simulink model "traj_controller_mass_point_example"  (R2018b)
settings: Solver=ode1  StartTime=0.0  StopTime=80  FixedStep=0.001  RelTol=1e-3
values from neighbouring files (symbols this model uses):
  cycle = true    [traj_controller_mass_point_example_init.m]    (also in traj_from_waypoints_example.m = false; traj_rigid_body_example_init.m)
  inital_velo = 8    [traj_controller_mass_point_example_init.m]    (also in traj_from_waypoints_example.m = 15; traj_rigid_body_example_init.m = 20)
  traj = trajFromWaypoints(traj_empty, waypoints, degree, cycle)    [traj_controller_mass_point_example_init.m]    (also in traj_from_waypoints_example.m = trajFromWaypoints(traj, waypoints, degree, cycle); traj_rigid_body_example_init.m)
  waypoints = [1 -1 0.2; 2 0 0.1; 1 1 0; -1 -1 0; -2 0 0.1; -1 1 0.2]'*50    [traj_controller_mass_point_example_init.m]    (also in traj_from_waypoints_example.m = [1 1 1; 2 2 2; 3 3 3; 4 4 4]'; traj_rigid_body_example_init.m)
libraries: actuators_lib x2, rigidBody_lib x1, simulink x1, traj_lib x1
settings Model: Creator=Fgücker  LastModifiedBy=yannic

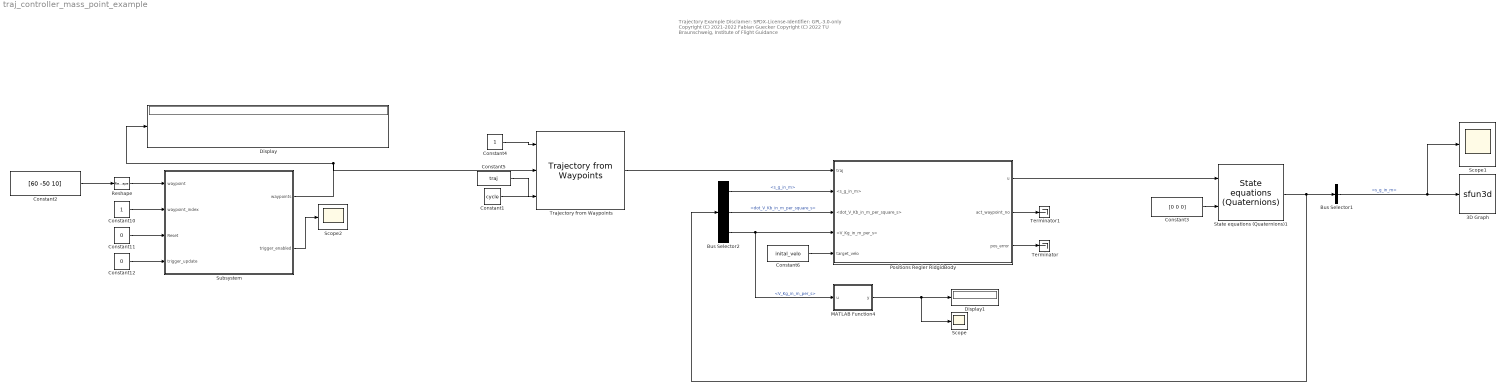
== system traj_controller_mass_point_example ==
  note: Trajectory Example
      |
      | Disclamer:
      | SPDX-License-Identifier: GPL-3.0-only
      |
      | Copyright (C) 2021-2022 Fabian Guecker
      | Copyright (C) 2022 TU Braunschweig, Institute of Flight Guidance
  3D Graph : S-Function  LoadFcn=if exist('sfun3d','file'), sfun3d([],[],[],'LoadBlock'); end  FunctionName=sfun3d  Parameters=ax,T,np,cp,gd,ls,mk,mx,hd,tb  SFunctionDeploymentMode=off  EnableBusSupport=off  mask(3D Graph){np=1, ax=[-1 1 -1 1 -1 1]*300, mx=1e4, T=0.040, cp=[0 0 1]*20, gd=on, hd=off, tb=off, ls=-, mk=none}
      mask prompts: np "Number of moving points (lines)"; ax "Range: [xmin xmax  ymin ymax zmin zmax]"; mx "Max number of points in each line"; T "Sampling Time"; cp "Camera position (use [0 0 1] for 2D XY view)"; gd "Grid (on|off)"; hd "HeadMarkers (on|off)"; tb "Toolbar (on|off)"; ls "LineStyle"; mk "LineMarker"
      mask help:
      | This block plots the position of several points in the XYZ space. The input contains the coordinates of all the points (x1,y1,z1,x2,y2,z2,...).
      | The number of moving points (lines), the XYZ ranges, sampling time, camera position, and grid (among other things) can be set as mask parameters.
      settings: CopyFcn=if exist('sfun3d','file'), sfun3d([],[],[],'CopyBlock'); end  DeleteFcn=if exist('sfun3d','file'), sfun3d([],[],[],'DeleteBlock'); end  NameChangeFcn=if exist('sfun3d','file'), sfun3d([],[],[],'NameChange'); end
      mask Help:
      | This block plots the position of several points in the XYZ space. The input contains the coordinates of all the points (x1,y1,z1,x2,y2,z2,...).
      | The number of moving points (lines), the XYZ ranges, sampling time, camera position, and grid (among other things) can be set as mask parameters.
      mask TypeOptions ls: - | -- | : | -. | none
      mask TypeOptions mk: none | . | + | o | * | x | square | diamond | v | ^ | > | < | pentagram | hexagram
      mask Display: plot([.05 .95 .95 .05 .05],[.45 .45 .95 .95 .45], 0.5+cos(0:0.1:2*pi)*0.3,0.7+sin(0:0.1:2*pi)*0.2)
  Bus Selector1 : BusSelector  OutputSignals=s_g_in_m
  Bus Selector2 : BusSelector  OutputSignals=s_g_in_m,dot_V_Kb_in_m_per_square_s,V_Kg_in_m_per_s
  Constant1 : Constant  Value=cycle  OutDataTypeStr=boolean
  Constant10 : Constant
  Constant11 : Constant  Value=0
  Constant12 : Constant  Value=0
  Constant2 : Constant  Value=[60 -50 10]
  Constant3 : Constant  Value=[0 0 0]
  Constant4 : Constant  OutDataTypeStr=boolean
  Constant5 : Constant  Value=traj  OutDataTypeStr=Bus: trajectoryBus
  Constant6 : Constant  Value=inital_velo
  Display : Display
  Display1 : Display
  MATLAB Function4 : MATLAB Function  TreatAsAtomicUnit=on
  Positions Regler RidgidBody : Subsystem
  Reshape : Reshape  OutputDimensionality=Column vector (2-D)
  Scope : Scope
  Scope1 : Scope
  Scope2 : Scope
  State equations (Quaternions)1 : rigidBody_lib/State equations (Quaternions)  m=1  I=eye(3)  g=9.81  omega_Kb_0=[0,0,0]'  q_bg_0=[1,0,0,0]'  V_Kb_0=inital_vel_vec  s_g_0=inital_point
  Subsystem : Subsystem  mask{MaxNumWaypoints=6}
      mask prompts: MaxNumWaypoints "Max. number of waypoints"
  Terminator : Terminator
  Terminator1 : Terminator
  Trajectory from Waypoints : traj_lib/Trajectory from Waypoints  traj_params=traj_params
      settings: SourceProductName=LADAC
  wires:
  Constant3/1 -> State equations (Quaternions)1/2
  State equations (Quaternions)1/1 -> Bus Selector1/1, Bus Selector2/1
  Bus Selector1/1 -> Scope1/1, 3D Graph/1  "<s_g_in_m>"
  Constant2/1 -> Reshape/1
  Subsystem/2(trigger_enabled) -> Scope2/1
  Subsystem/1(waypoints) -> Trajectory from Waypoints/2, Display/1
  Constant10/1 -> Subsystem/2(waypoint_index)
  Constant11/1 -> Subsystem/3(Reset)
  Constant12/1 -> Subsystem/4(trigger_update)
  Constant4/1 -> Trajectory from Waypoints/1
  Trajectory from Waypoints/1 -> Positions Regler RidgidBody/1(traj)
  Bus Selector2/1 -> Positions Regler RidgidBody/2(<s_g_in_m>)  "<s_g_in_m>"
  Bus Selector2/2 -> Positions Regler RidgidBody/3(<dot_V_Kb_in_m_per_square_s>)  "<dot_V_Kb_in_m_per_square_s>"
  Bus Selector2/3 -> MATLAB Function4/1(u), Positions Regler RidgidBody/4(<V_Kg_in_m_per_s>)  "<V_Kg_in_m_per_s>"
  Positions Regler RidgidBody/1(u) -> State equations (Quaternions)1/1
  Constant6/1 -> Positions Regler RidgidBody/5(target_velo)
  Positions Regler RidgidBody/3(pos_error) -> Terminator/1
  Positions Regler RidgidBody/2(act_waypoint_no) -> Terminator1/1
  MATLAB Function4/1(y) -> Scope/1, Display1/1
  Reshape/1 -> Subsystem/1(waypoint)
  Constant1/1 -> ?
  Constant5/1 -> Trajectory from Waypoints/3

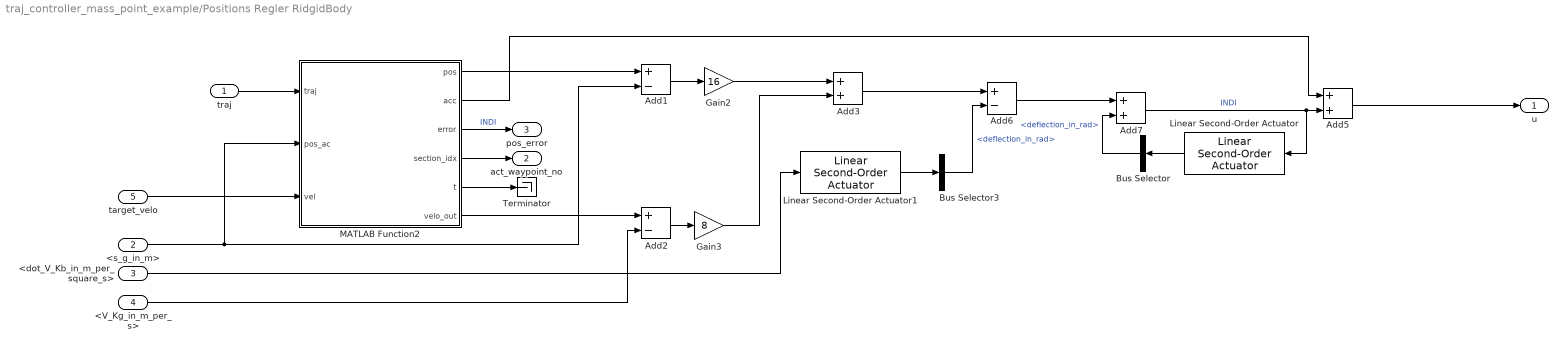
== system traj_controller_mass_point_example/Positions Regler RidgidBody ==
  traj : Inport
  <s_g_in_m> : Inport  Port=2
  <dot_V_Kb_in_m_per_square_s> : Inport  Port=3
  <V_Kg_in_m_per_s> : Inport  Port=4
  target_velo : Inport  Port=5
  Add1 : Sum  Inputs=+-
  Add2 : Sum  Inputs=+-
  Add3 : Sum
  Add5 : Sum
  Add6 : Sum  Inputs=+-
  Add7 : Sum
  Bus Selector : BusSelector  OutputSignals=deflection_in_rad
  Bus Selector3 : BusSelector  OutputSignals=deflection_in_rad
  Gain2 : Gain  Gain=16
  Gain3 : Gain  Gain=8
  Linear Second-Order Actuator : actuators_lib/Linear Second-Order Actuator  omega=40  d=1  A_0=0  dot_A_0=0  start_steady_state=off
      settings: SourceProductName=LADAC
  Linear Second-Order Actuator1 : actuators_lib/Linear Second-Order Actuator  omega=80  d=1  A_0=0  dot_A_0=0  start_steady_state=off
      settings: SourceProductName=LADAC
  MATLAB Function2 : MATLAB Function  TreatAsAtomicUnit=on
  Terminator : Terminator
  u : Outport
  act_waypoint_no : Outport  Port=2
  pos_error : Outport  Port=3
  wires:
  Add1/1 -> Gain2/1
  MATLAB Function2/6(velo_out) -> Add2/1
  Bus Selector3/1 -> Add6/2  "<deflection_in_rad>"
  Add5/1 -> u/1
  MATLAB Function2/5(t) -> Terminator/1
  Gain2/1 -> Add3/1
  Add3/1 -> Add6/1
  Add7/1 -> Linear Second-Order Actuator/1, Add5/2  "INDI"
  Bus Selector/1 -> Add7/2  "<deflection_in_rad>"
  <s_g_in_m>/1 -> Add1/2, MATLAB Function2/2(pos_ac)
  <V_Kg_in_m_per_s>/1 -> Add2/2
  Linear Second-Order Actuator1/1 -> Bus Selector3/1
  MATLAB Function2/1(pos) -> Add1/1
  Linear Second-Order Actuator/1 -> Bus Selector/1
  MATLAB Function2/2(acc) -> Add5/1
  <dot_V_Kb_in_m_per_square_s>/1 -> Linear Second-Order Actuator1/1
  traj/1 -> MATLAB Function2/1(traj)
  MATLAB Function2/3(error) -> pos_error/1  "INDI"
  Gain3/1 -> Add3/2
  MATLAB Function2/4(section_idx) -> act_waypoint_no/1
  Add2/1 -> Gain3/1
  Add6/1 -> Add7/1
  target_velo/1 -> MATLAB Function2/3(vel)

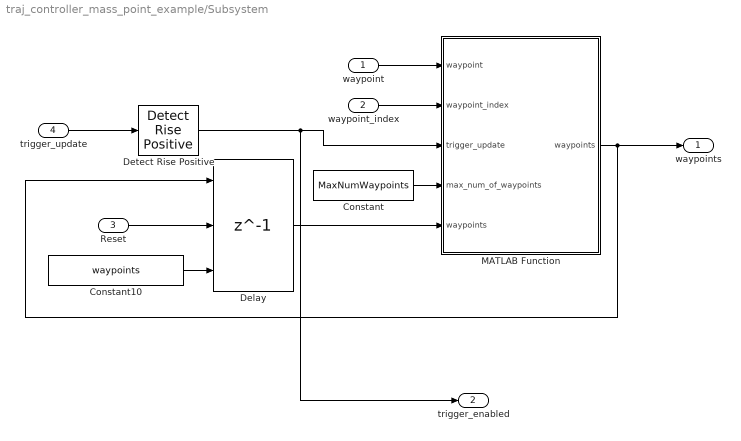
== system traj_controller_mass_point_example/Subsystem ==
  waypoint : Inport
  waypoint_index : Inport  Port=2
  Reset : Inport  Port=3
  trigger_update : Inport  Port=4
  Constant : Constant  Value=MaxNumWaypoints
  Constant10 : Constant  Value=waypoints
  Delay : Delay  DelayLength=1  InitialConditionSource=Input port  ExternalReset=Rising
      settings: InputPortMap=u0,r5,p4
  Detect Rise Positive : simulink/Logic and Bit Operations/Detect Rise Positive  vinit=0  OutDataTypeStr=boolean
  MATLAB Function : MATLAB Function  TreatAsAtomicUnit=on
  waypoints : Outport
  trigger_enabled : Outport  Port=2
  wires:
  Constant10/1 -> Delay/3
  MATLAB Function/1(waypoints) -> Delay/1, waypoints/1
  Reset/1 -> Delay/2
  waypoint_index/1 -> MATLAB Function/2(waypoint_index)
  Delay/1 -> MATLAB Function/5("waypoints ")
  waypoint/1 -> MATLAB Function/1(waypoint)
  Detect Rise Positive/1 -> trigger_enabled/1, MATLAB Function/3(trigger_update)
  Constant/1 -> MATLAB Function/4(max_num_of_waypoints)
  trigger_update/1 -> Detect Rise Positive/1

== matlab function traj_controller_mass_point_example/Subsystem/MATLAB Function ==
  data: waypoints output; waypoint input; waypoint_index input; trigger_update input; max_num_of_waypoints input; waypoints input
function waypoints = fcn(waypoint, waypoint_index, trigger_update, max_num_of_waypoints, waypoints)

if(trigger_update)
    if(waypoint_index >= 1) && (waypoint_index <= max_num_of_waypoints)
        waypoints(:,waypoint_index) = waypoint;
    end
end

end

== matlab function traj_controller_mass_point_example/Positions Regler RidgidBody/MATLAB Function2 ==
  data: pos output; acc output; traj input; pos_ac input; vel input; error output; section_idx output; t output; velo_out output
function [pos, acc, error,section_idx, t, velo_out]  = GetMatch(traj, pos_ac, vel)

section_idx = 1;

[section_idx, error, t] = trajGetMatch(traj, pos_ac, section_idx);

active_section = trajGetSection(traj, section_idx);

pos = trajSectionGetPos(active_section, t);

acc = trajSectionGetAcc(active_section, vel, t);

[T] = trajSectionGetFrenetSerret(active_section, t);

% Replace NaNs with zero
T(isnan(T)) = 0;

velo_out = T * vel;

end

== matlab function traj_controller_mass_point_example/MATLAB Function4 ==
  data: u input; y output
function y = fcn(u)

y = norm(u);
